simulink model "IPMSMVelocityControl"  (R2024a)
settings: Solver=FixedStepDiscrete  StartTime=0.0  StopTime=1  FixedStep=Ts  RelTol=1e-3  EnableMultiTasking=on
PreLoadFcn:
  | IPMSMVelocityControlData;
undefined symbols (not defined in the file): Ld, Lq, p, psim, Ts, VDC_VECT
libraries: nesl_utility x13, fl_lib x10, ee_lib x4, eeTransforms x2, batteryecm_lib x1, eePmsmCurrentController x1, simulink x1, eePmsmCurrentReferenceGen x1, eeVelocityController x1, eePwmGeneratorTwoLevel x1, SignalEditorBlockLib x1
CloseFcn:
  | try,close(h1_IPMSMVelocityControl),end
  | clear h1_IPMSMVelocityControl
  | 
  | clear simlog_IPMSMVelocityControl
  | clear logsout_IPMSMVelocityControl
  | 
  | clear Pmax Tmax p psim Ld Lq L0 Rs Jm
  | clear Cdc Vnom V1 AH0
  | clear Ts fsw Tsi Tso Kp_id Ki_id Kp_iq Ki_iq
  | clear numd_id dend_id numd_iq dend_iq
  | clear Kp_omega Ki_omega numd_omega dend_omega
  | clear ID_MAP IQ_MAP RPM_VECT TQ_VECT VDC_VECT
Description:
  | IPMSM Velocity Control
settings Model: Creator=The MathWorks, Inc.  LastModifiedBy=hirah
settings SolverCC: AlgebraicLoopSolver=TrustRegion  MaxZcPerStep=1
settings DataIOCC: MaxDataPoints=210000  ReturnWorkspaceOutputs=off  SignalLoggingName=logsout_IPMSMVelocityControl
settings OptimizationCC: ReuseModelBlockBuffer=off  LifeSpan=inf
settings DebuggingCC: UnderspecifiedInitializationDetection=Classic  MergeDetectMultiDrivingBlocksExec=none  UnconnectedInputMsg=warning  UnconnectedOutputMsg=warning  UnconnectedLineMsg=warning  SFUnexpectedBacktrackingDiag=warning  SFNoUnconditionalDefaultTransitionDiag=warning  SFExecutionAtInitializationDiag=none  ArithmeticOperatorsInVariantConditions=warning
settings ModelReferenceCC: EnableRefExpFcnMdlSchedulingChecks=on
settings SFSimCC: SimUseLocalCustomCode=off  CustomCodeUndefinedFunction=UseInterfaceOnly
settings RTWCC: RTWUseLocalCustomCode=off  GPUComputeCapability=3.5  DLArmComputeVersion=19.05
settings CodeAppCC: StateflowObjectComments=on
settings GRTTargetCC: TargetLangStandard=C89/C90 (ANSI)
settings ConfigComp: CovMetricSettings=dw  CovSaveCumulativeToWorkspaceVar=on  CovSaveSingleToWorkspaceVar=on  CovExternalEMLEnable=off
settings SimscapeCC: SimscapeNormalizeSystem=off  SimscapeLogType=all  SimscapeLogSimulationStatistics=on  SimscapeLogName=simlog_IPMSMVelocityControl  SimscapeLogDataHistory=210000

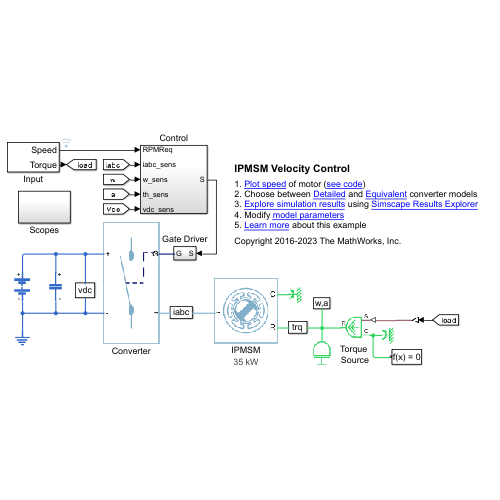
[thumbnail: Simulink's stored preview of the top-level diagram]
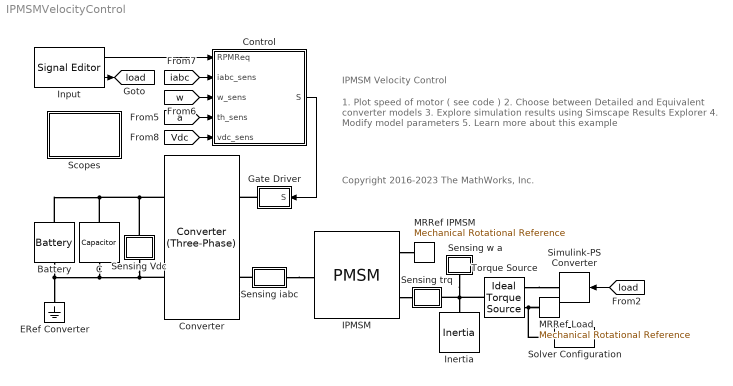
== system IPMSMVelocityControl ==
  note: IPMSM Velocity Control
  note: 1. Plot speed of motor ( see code )
      | 2. Choose between Detailed and Equivalent converter models
      | 3. Explore simulation results using Simscape Results Explorer
      | 4. Modify model parameters
      | 5. Learn more about this example
  note: Copyright 2016-2023 The MathWorks, Inc.
  Battery : batteryecm_lib/Battery  Vnom=Vnom V  prm_dir=1  R1_dis=2 Ohm  R1_ch=2 Ohm  R1=0.001 Ohm  prm_AH=1  AH=300 hr*A  V1=V1 V  AH1=100 hr*A  prm_R2=1  R2=2000 Ohm  Tmeas=298.15 K  charge_measurement_port=simscape.enum.battery.enable.no  prm_dyn=1  Rp1=0.005 Ohm  tau1=30 s  Rp2=0.005 Ohm  tau2=30 s  Rp3=0.005 Ohm  tau3=30 s  Rp4=0.005 Ohm  tau4=30 s  Rp5=0.005 Ohm  tau5=30 s  prm_fade=1  N_fade=100  AH_fade=45 hr*A  R1_fade=2.02 Ohm  R1_ch_fade=2.02 Ohm  V1_fade=10.35 V  prm_age=1  prm_age_OCV=1  OCV_age=0.9  SOC_age=60  Tmeas_age=298.15 K  delta_time_age_vec=[0] d  temperature_age_vec=[273] K  OCV_scaling_age=2.2134e6  OCV_offset_age=1.632e6  temp_exp_age=0.515833569 V  t_exp_age=0.75  Vnom_T2=12 V  R1_T2=2.2 Ohm  R1_T2_dis=2.2 Ohm  R1_T2_ch=2.2 Ohm  V1_T2=11.4 V  R2_T2=2200 Ohm  Rp1_T2=0.005 Ohm  tau1_T2=30 s  Rp2_T2=0.005 Ohm  tau2_T2=30 s  Rp3_T2=0.005 Ohm  tau3_T2=30 s  Rp4_T2=0.005 Ohm  tau4_T2=30 s  Rp5_T2=0.005 Ohm  tau5_T2=30 s  Tmeas2=273.15 K  thermal_port=simscape.enum.thermaleffects.omit  thermal_mass=30000 J/K  i_specify=off  i_priority=None  i=0 A  i_nominal_specify=off  i_nominal_value=1  i_nominal_unit=A  v_specify=off  v_priority=None  v=0 V  v_nominal_specify=off  v_nominal_value=1  v_nominal_unit=V  charge_specify=on  charge_priority=High  charge=AH0 hr*A  charge_nominal_specify=off  charge_nominal_value=1  charge_nominal_unit=A*hr  num_cycles_specify=off  num_cycles_priority=High  num_cycles=0  num_cycles_nominal_specify=off  num_cycles_nominal_value=1  num_cycles_nominal_unit=1  temperature_specify=off  temperature_priority=High  temperature=298.15 K  temperature_nominal_specify=off  temperature_nominal_value=1  temperature_nominal_unit=K
  C : fl_lib/Electrical/Electrical Elements/Capacitor  c=Cdc F  r=1e-6 Ohm  g=0 1/Ohm  i_specify=off  i_priority=None  i=0 A  i_nominal_specify=off  i_nominal_value=1  i_nominal_unit=A  v_specify=off  v_priority=None  v=0 V  v_nominal_specify=off  v_nominal_value=1  v_nominal_unit=V  vc_specify=on  vc_priority=None  vc=Vnom V  vc_nominal_specify=off  vc_nominal_value=1  vc_nominal_unit=V
  Control : Subsystem
  Converter : ee_lib/Semiconductors & Converters/Converters/Converter (Three-Phase)  port_option=ee.enum.threePhasePort.composite  fidelity_option=ee.enum.converters.fidelity.detailed  device_type=3  K=0  Vf=0.8 V  Ron=0.001 Ohm  Rds=0.001 Ohm  Goff=1e-5 1/Ohm  Vgt=1 V  Vgt_off=-1 V  Ih=1 A  Vth=0.5 V  diode_param=2  diode_Vf=0.8 V  diode_Ron=0.001 Ohm  diode_Goff=1e-5 1/Ohm  diode_C=50 nF  diode_iRM=-235 A  diode_iF=300 A  diode_idot=-50 A/us  diode_trr_param=1  diode_trr_factor=3  diode_trr=15 us  diode_Qrr=1.5e+3 s*uA  snubber_type=0  Cs=1e-7 F  Rs=0.1 Ohm
  ERef Converter : fl_lib/Electrical/Electrical Elements/Electrical Reference
  Gate Driver : Subsystem
  IPMSM : ee_lib/Electromechanical/Permanent Magnet/PMSM  port_option=ee.enum.threePhasePort.composite  winding_type=ee.enum.statorconnection.wye  machine_param=ee.enum.pmsm.parameterization.constant  nPolePairs=p  pmflux_param=1  pm_flux_linkage=psim Wb  torque_constant=0.18 N*m/A  back_emf_constant=0.18 V/(rad/s)  stator_param=1  Ld=Ld H  Lq=Lq H  idVec=[-200, 0, 200] A  iqVec=[-200, 0, 200] A  LdMatrix=0.0002 * ones(3, 3) H  LqMatrix=0.0002 * ones(3, 3) H  PmMatrix=0.1 * ones(3, 3) Wb  ktMatrix=0.18 * ones(3, 3) N*m/A  keMatrix=0.18 * ones(3, 3) V/(rad/s)  L0=L0 H  Ls=0.0002 H  Lm=0.00002 H  Ms=0.00002 H  Rs=Rs Ohm  zero_sequence=ee.enum.park.zerosequence.exclude  axes_param=1  loss_param=ee.enum.ironloss.none  losses_oc=[0, 0, 0] W  losses_sc=[0, 0, 0] W  f_losses=60 Hz  Isc_losses=95 A  J=0 kg*m^2  lam=0 N*m/(rad/s)  i_d_specify=off  i_d_priority=None  i_d=0 A  i_d_nominal_specify=off  i_d_nominal_value=1  i_d_nominal_unit=A  i_q_specify=off  i_q_priority=None  i_q=0 A  i_q_nominal_specify=off  i_q_nominal_value=1  i_q_nominal_unit=A  torque_specify=off  torque_priority=None  torque=0 N*m  torque_nominal_specify=off  torque_nominal_value=1  torque_nominal_unit=N*m  angular_velocity_specify=on  angular_velocity_priority=None  angular_velocity=0 rpm  angular_velocity_nominal_specify=off  angular_velocity_nominal_value=1  angular_velocity_nominal_unit=rpm  angular_position_specify=on  angular_position_priority=High  angular_position=0 rad  angular_position_nominal_specify=off  angular_position_nominal_value=1  angular_position_nominal_unit=deg  alpha=3.93e-3 1/K  alpha_flux=-0.001 1/K  Tmeas=298.15 K  stator_thermal_mass=100 J/K  rotor_thermal_mass=200 J/K  Rm_percent_rotor=90  Rd_percent_rotor=30  temperatureA_specify=off  temperatureA_priority=High  temperatureA=25 degC  temperatureA_nominal_specify=off  temperatureA_nominal_value=1  temperatureA_nominal_unit=degC  temperatureB_specify=off  temperatureB_priority=High  temperatureB=25 degC  temperatureB_nominal_specify=off  temperatureB_nominal_value=1  temperatureB_nominal_unit=degC  temperatureC_specify=off  temperatureC_priority=High  temperatureC=25 degC  temperatureC_nominal_specify=off  temperatureC_nominal_value=1  temperatureC_nominal_unit=degC  temperatureR_specify=off  temperatureR_priority=High  temperatureR=25 degC  temperatureR_nominal_specify=off  temperatureR_nominal_value=1  temperatureR_nominal_unit=degC
      settings: AttributesFormatString=35 kW  InternalSimscapePortConfiguration="{\"Bottom\":[],\"Left\":[{\"id\":\"N\",\"label\":\"~\",\"type\":\"foundation.electrical.three_phase\"}],\"Right\":[{\"id\":\"R\",\"label\":\"R\",\"type\":\"foundation.mechanical.rotational.rotational\"},{\"id\":\"C\",\"label\":\"C\",\"type\":\"foundation.mechanical.rotational.rotational\"}],\"Top\":[]}"
  Inertia : fl_lib/Mechanical/Rotational Elements/Inertia  inertia=Jm kg*m^2  num_ports=foundation.enum.numPorts2.one  w_specify=on  w_priority=High  w=0 rpm  w_nominal_specify=off  w_nominal_value=1  w_nominal_unit=rad/s  t_specify=off  t_priority=High  t=0 N*m  t_nominal_specify=off  t_nominal_value=1  t_nominal_unit=N*m
  Input : SignalEditorBlockLib/Signal Editor  FileName=IPMSMVelocityControlInput.mat  ActiveScenario=Test_1  ActiveSignal=Torque  IsBus=off  OutputBusObjectStr=Bus: BusObject  SampleTime=0  OutputAfterFinalValue=Extrapolation  Unit=inherit  PreserveSignalName=on  ApplySigPropsToAllScenarios=on  ApplySigPropsToAllSignals=off
  MRRef IPMSM : fl_lib/Mechanical/Rotational Elements/Mechanical Rotational Reference
  MRRef Load : fl_lib/Mechanical/Rotational Elements/Mechanical Rotational Reference
  Scopes : Subsystem
  Sensing Vdc : Subsystem
      mask Display: disp('vdc')
  Sensing trq : Subsystem
      mask Display: disp('trq')
  Sensing w a : Subsystem
      mask Display: disp('w,a')
  Sensing iabc : Subsystem
      mask Display: disp('iabc')
  Simulink-PS Converter : nesl_utility/Simulink-PS Converter  PhysicalDomain=network_engine_domain  SubClassName=ps_input  LeftPortType=input  RightPortType=output  PseudoPeriodic=off  Frequencies=[]  NoiseDistribution=none  NoiseParameters=[]  Unit=N*m  AffineConversion=off  FilteringAndDerivatives=zero  SimscapeFilterOrder=1  InputFilterTimeConstant=0.001  UdotUserProvided=1
  Solver Configuration : nesl_utility/Solver Configuration  PhysicalDomain=network_engine_domain  SubClassName=solver  LeftPortType=input  RightPortType=generic  Tones=[]  Harmonics=[]  SimulateNoise=off  Profile=off  UseLocalSampling=off  EnableSwitchedLinearOptims=on  FrequencyDomain=off  UseCCode=off  RelTol=0.001  AbsTol=1e-06  MinStep=1e-09  ToWorkspace=off  RevertToSquareIcSolve=off  NumHomotopyIterations=100  PhasorMode=off  PhasorModeNumHarmonics=1  ConsistencySolver=NEWTON_FTOL  IndexReductionMethod=DerivativeReplacement  DoDC=off  ResidualTolerance=1e-9  ConsistencyTolSource=GLOBAL  ConsistencyAbsTol=0.001  ConsistencyRelTol=0.001  ConsistencyTolFactor=0.001  UseLocalSolver=on  LocalSolverChoice=NE_BACKWARD_EULER_ADVANCER  ResolveIndetEquations=on  FunctionEvalNumThread=1  LocalSolverSampleTime=Ts  DoFixedCost=on  MaxNonlinIter=5  MaxModeIter=2  ComputeImpulses=off  ImpulseIterations=2  LinearAlgebra=auto  LinearAlgebraNumThread=0  EquationFormulation=NE_TIME_EF  DelaysMemoryBudget=1024  AutomaticFiltering=on  FilteringTimeConstant=0.001  PartitionStorageMethod=AS_NEEDED  PartitionMemoryBudget=1024  PartitionMethod=FAST  MultibodyUseLocalSolver=off  MultibodyLocalSolverChoice=ODE1  MultibodyLocalSolverSampleTime=0.001
  Torque Source : fl_lib/Mechanical/Mechanical Sources/Ideal Torque Source
  tag scope: load=global
  wires:
  Control/1(S) -> Gate Driver/1(S)
  [load] -> Simulink-PS Converter/1
  Input/1 -> Control/1(RPMReq)
  [Vdc] -> Control/5(vdc_sens)
  [iabc] -> Control/2(iabc_sens)
  [w] -> Control/3(w_sens)
  [a] -> Control/4(th_sens)
  Input/2 -> [load]
  connections:
  Converter/RConn1 -- Sensing Vdc/LConn1 -- Battery/LConn1 -- C/LConn1
  Torque Source/LConn1 -- Sensing trq/RConn1 -- Inertia/LConn1 -- Sensing w a/LConn1
  Gate Driver/RConn1 -- Converter/LConn1
  Torque Source/RConn1 -- Simulink-PS Converter/RConn1
  Torque Source/RConn2 -- Solver Configuration/RConn1 -- MRRef Load/LConn1
  Sensing iabc/LConn1 -- Converter/LConn2
  Sensing iabc/RConn1 -- IPMSM/LConn1
  IPMSM/RConn2 -- MRRef IPMSM/LConn1
  IPMSM/RConn1 -- Sensing trq/LConn1
  Battery/RConn1 -- Converter/RConn2 -- Sensing Vdc/RConn1 -- C/RConn1 -- ERef Converter/LConn1

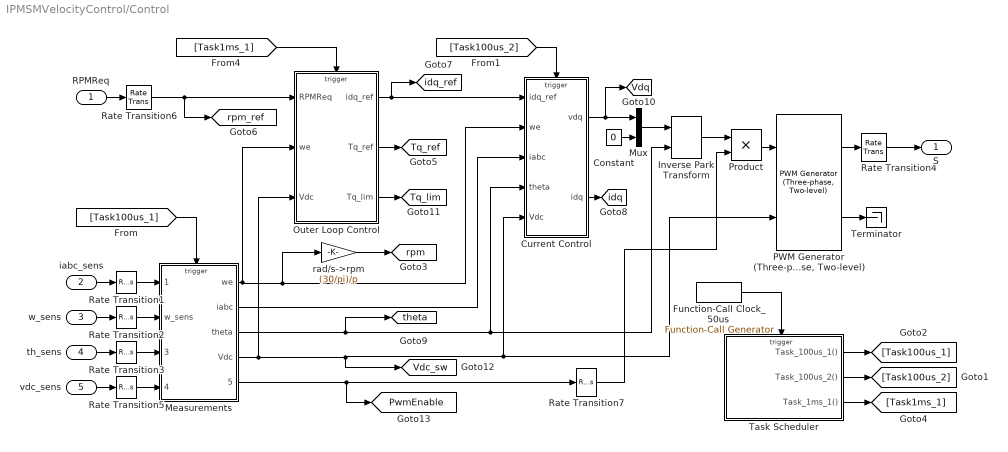
== system IPMSMVelocityControl/Control ==
  RPMReq : Inport
  iabc_sens : Inport  Port=2
  w_sens : Inport  Port=3
  th_sens : Inport  Port=4
  vdc_sens : Inport  Port=5
  Constant : Constant  Value=0  SampleTime=-1
  Current Control : Subsystem
  Function-Call Clock_50us : simulink/Ports & Subsystems/Function-Call Generator  sample_time=5e-5  numberOfIterations=1  DisallowWideOutput=off
  Inverse Park Transform : eeTransforms/Inverse Park Transform  AxisAlignment=Q-axis  PowerInvariant=off
  Measurements : Subsystem
  Mux : Mux  Inputs=2
  Outer Loop Control : Subsystem
  "PWM Generator (Three-phase, Two-level)" : eePwmGeneratorTwoLevel/PWM Generator (Three-phase, Two-level)  PWMMode=Continuous PWM (CPWM)  CPWMMode=SVM: space vector modulation  DPWMMode=60 DPWM: 60 degree discontinuous PWM  fsw=fsw  Ts=Ts
  Product : Product
  Rate Transition{1..7} (7 alike) : RateTransition
  Task Scheduler : Stateflow chart  TreatAsAtomicUnit=on
  Terminator : Terminator
  rad/s->rpm : Gain  Gain=(30/pi)/p
  S : Outport  VectorParamsAs1DForOutWhenUnconnected=off
  tag scope: PwmEnable=global, Tq_lim=global, Tq_ref=global, Vdc_sw=global, Vdq=global, idq=global, idq_ref=global, rpm=global, rpm_ref=global, theta=global
  wires:
  [Task100us_1] -> Measurements/Trigger
  [Task100us_2] -> Current Control/Trigger
  Current Control/1(vdq) -> Mux/1, [Vdq]
  Measurements/2(iabc) -> Current Control/3(iabc)
  Measurements/3(theta) -> [theta], Current Control/4(theta), Inverse Park Transform/2
  "PWM Generator (Three-phase, Two-level)"/1 -> Rate Transition4/1
  iabc_sens/1 -> Rate Transition1/1
  w_sens/1 -> Rate Transition2/1
  th_sens/1 -> Rate Transition3/1
  vdc_sens/1 -> Rate Transition5/1
  Outer Loop Control/1(idq_ref) -> [idq_ref], Current Control/1(idq_ref)
  RPMReq/1 -> Rate Transition6/1
  "PWM Generator (Three-phase, Two-level)"/2 -> Terminator/1
  Rate Transition1/1 -> Measurements/1(iabc_sens)
  Rate Transition2/1 -> Measurements/2(w_sens)
  Rate Transition3/1 -> Measurements/3(th_sens)
  Rate Transition5/1 -> Measurements/4(Vdc_sens)
  Rate Transition6/1 -> [rpm_ref], Outer Loop Control/1(RPMReq)
  Measurements/4(Vdc) -> [Vdc_sw], Current Control/5(Vdc), "PWM Generator (Three-phase, Two-level)"/2, Outer Loop Control/3(Vdc)
  Function-Call Clock_50us/1 -> Task Scheduler/Trigger
  Task Scheduler/3(Task_1ms_1()) -> [Task1ms_1]
  Task Scheduler/2(Task_100us_2()) -> [Task100us_2]
  Task Scheduler/1(Task_100us_1()) -> [Task100us_1]
  Outer Loop Control/2(Tq_ref) -> [Tq_ref]
  Measurements/1(we) -> Current Control/2(we), rad/s->rpm/1, Outer Loop Control/2(we)
  rad/s->rpm/1 -> [rpm]
  Current Control/2(idq) -> [idq]
  Outer Loop Control/3(Tq_lim) -> [Tq_lim]
  Measurements/5(PwmEnable) -> [PwmEnable], Rate Transition7/1
  [Task1ms_1] -> Outer Loop Control/Trigger
  Mux/1 -> Inverse Park Transform/1
  Constant/1 -> Mux/2
  Rate Transition4/1 -> S/1
  Product/1 -> "PWM Generator (Three-phase, Two-level)"/1
  Inverse Park Transform/1 -> Product/1
  Rate Transition7/1 -> Product/2

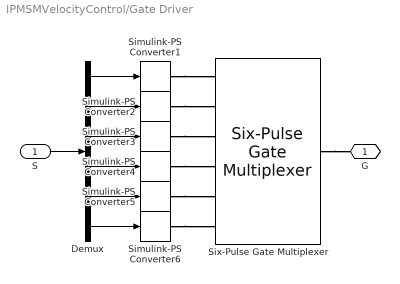
== system IPMSMVelocityControl/Gate Driver ==
  S : Inport
  Demux : Demux  Outputs=6
  Simulink-PS Converter{1..6} (6 alike) : nesl_utility/Simulink-PS Converter  PhysicalDomain=network_engine_domain  SubClassName=ps_input  LeftPortType=input  RightPortType=output  PseudoPeriodic=off  Frequencies=[]  NoiseDistribution=none  NoiseParameters=[]  Unit=1  AffineConversion=off  FilteringAndDerivatives=zero  SimscapeFilterOrder=1  InputFilterTimeConstant=0.001  UdotUserProvided=1
  Six-Pulse Gate Multiplexer : ee_lib/Semiconductors & Converters/Converters/Six-Pulse Gate Multiplexer  port_option=ee.enum.controlport.ps
  G : PMIOPort  Side=Right
  wires:
  Demux/1 -> Simulink-PS Converter1/1
  S/1 -> Demux/1
  Demux/4 -> Simulink-PS Converter4/1
  Demux/2 -> Simulink-PS Converter2/1
  Demux/3 -> Simulink-PS Converter3/1
  Demux/5 -> Simulink-PS Converter5/1
  Demux/6 -> Simulink-PS Converter6/1
  connections:
  Six-Pulse Gate Multiplexer/RConn1 -- G/RConn1
  Simulink-PS Converter1/RConn1 -- Six-Pulse Gate Multiplexer/LConn1
  Simulink-PS Converter3/RConn1 -- Six-Pulse Gate Multiplexer/LConn3
  Simulink-PS Converter5/RConn1 -- Six-Pulse Gate Multiplexer/LConn5
  Simulink-PS Converter6/RConn1 -- Six-Pulse Gate Multiplexer/LConn6
  Simulink-PS Converter4/RConn1 -- Six-Pulse Gate Multiplexer/LConn4
  Simulink-PS Converter2/RConn1 -- Six-Pulse Gate Multiplexer/LConn2

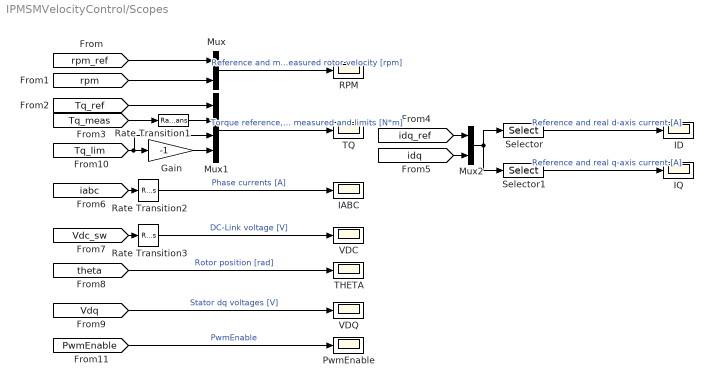
== system IPMSMVelocityControl/Scopes ==
  Gain : Gain  Gain=-1
  IABC : Scope
  ID : Scope
  IQ : Scope
  Mux : Mux  Inputs=2
  Mux1 : Mux
  Mux2 : Mux  Inputs=2
  PwmEnable : Scope
  RPM : Scope
  Rate Transition1 : RateTransition
  Rate Transition2 : RateTransition  OutPortSampleTime=1e-4
  Rate Transition3 : RateTransition  OutPortSampleTime=1e-4
  Selector : Selector  InputPortWidth=4  IndexOptions=Index vector (dialog)  Indices=[1 3]  OutputSizes=1
  Selector1 : Selector  InputPortWidth=4  IndexOptions=Index vector (dialog)  Indices=[2 4]  OutputSizes=1
  THETA : Scope
  TQ : Scope
  VDC : Scope
  VDQ : Scope
  wires:
  [rpm] -> Mux/2
  Selector1/1 -> IQ/1  "Reference and real q-axis current [A]"
  Mux2/1 -> Selector1/1, Selector/1
  Gain/1 -> Mux1/4
  Rate Transition3/1 -> VDC/1  "DC-Link voltage [V]"
  [Vdc_sw] -> Rate Transition3/1
  [idq_ref] -> Mux2/1
  [PwmEnable] -> PwmEnable/1  "PwmEnable"
  [Tq_ref] -> Mux1/1
  Rate Transition2/1 -> IABC/1  "Phase currents [A]"
  [idq] -> Mux2/2
  [rpm_ref] -> Mux/1
  [iabc] -> Rate Transition2/1
  [Tq_meas] -> Rate Transition1/1
  [Vdq] -> VDQ/1  "Stator dq voltages [V]"
  Selector/1 -> ID/1  "Reference and real d-axis current [A]"
  [Tq_lim] -> Mux1/3, Gain/1
  Mux1/1 -> TQ/1  "Torque reference, measured and limits [N*m]"
  [theta] -> THETA/1  "Rotor position [rad]"
  Rate Transition1/1 -> Mux1/2
  Mux/1 -> RPM/1  "Reference and measured rotor velocity [rpm]"

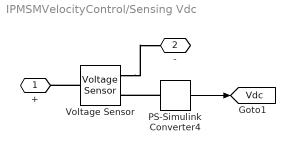
== system IPMSMVelocityControl/Sensing Vdc ==
  PS-Simulink Converter4 : nesl_utility/PS-Simulink Converter  PhysicalDomain=network_engine_domain  SubClassName=ps_output  LeftPortType=input  RightPortType=output  PseudoPeriodic=off  Frequencies=[]  VectorFormat=1-D array  Unit=V  AffineConversion=off
  Voltage Sensor : fl_lib/Electrical/Electrical Sensors/Voltage Sensor
  + : PMIOPort  Side=Left
  - : PMIOPort  Port=2  Side=Right
  tag scope: Vdc=global
  wires:
  PS-Simulink Converter4/1 -> [Vdc]
  connections:
  Voltage Sensor/LConn1 -- +/RConn1
  Voltage Sensor/RConn2 -- -/RConn1
  PS-Simulink Converter4/LConn1 -- Voltage Sensor/RConn1

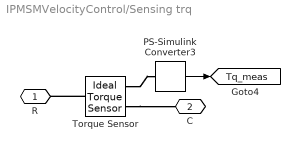
== system IPMSMVelocityControl/Sensing trq ==
  PS-Simulink Converter3 : nesl_utility/PS-Simulink Converter  PhysicalDomain=network_engine_domain  SubClassName=ps_output  LeftPortType=input  RightPortType=output  PseudoPeriodic=off  Frequencies=[]  VectorFormat=1-D array  Unit=N*m  AffineConversion=off
  Torque Sensor : fl_lib/Mechanical/Mechanical Sensors/Ideal Torque Sensor
  R : PMIOPort  Side=Left
  C : PMIOPort  Port=2  Side=Right
  tag scope: Tq_meas=global
  wires:
  PS-Simulink Converter3/1 -> [Tq_meas]
  connections:
  Torque Sensor/RConn1 -- C/RConn1
  Torque Sensor/RConn2 -- PS-Simulink Converter3/LConn1
  Torque Sensor/LConn1 -- R/RConn1

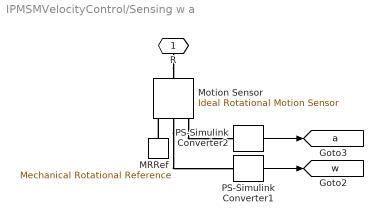
== system IPMSMVelocityControl/Sensing w a ==
  MRRef : fl_lib/Mechanical/Rotational Elements/Mechanical Rotational Reference
  Motion Sensor : fl_lib/Mechanical/Mechanical Sensors/Ideal Rotational Motion Sensor  reference=foundation.enum.MeasurementReference.difference  acceleration_port=false  velocity_port=true  position_port=true  wrap_angle=simscape.enum.onoff.off  offset=0 deg
  PS-Simulink Converter1 : nesl_utility/PS-Simulink Converter  PhysicalDomain=network_engine_domain  SubClassName=ps_output  LeftPortType=input  RightPortType=output  PseudoPeriodic=off  Frequencies=[]  VectorFormat=1-D array  Unit=rad/s  AffineConversion=off
  PS-Simulink Converter2 : nesl_utility/PS-Simulink Converter  PhysicalDomain=network_engine_domain  SubClassName=ps_output  LeftPortType=input  RightPortType=output  PseudoPeriodic=off  Frequencies=[]  VectorFormat=1-D array  Unit=rad  AffineConversion=off
  R : PMIOPort  Side=Left
  tag scope: a=global, w=global
  wires:
  PS-Simulink Converter1/1 -> [w]
  PS-Simulink Converter2/1 -> [a]
  connections:
  R/RConn1 -- Motion Sensor/LConn1
  Motion Sensor/RConn2 -- PS-Simulink Converter1/LConn1
  MRRef/LConn1 -- Motion Sensor/RConn1
  Motion Sensor/RConn3 -- PS-Simulink Converter2/LConn1

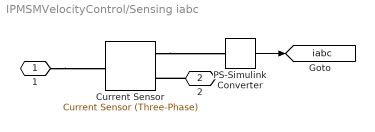
== system IPMSMVelocityControl/Sensing iabc ==
  Current Sensor : ee_lib/Sensors & Transducers/Current Sensor (Three-Phase)
  PS-Simulink Converter : nesl_utility/PS-Simulink Converter  PhysicalDomain=network_engine_domain  SubClassName=ps_output  LeftPortType=input  RightPortType=output  PseudoPeriodic=off  Frequencies=[]  VectorFormat=1-D array  Unit=A  AffineConversion=off
  1 : PMIOPort  Side=Left
  2 : PMIOPort  Port=2  Side=Right
  tag scope: iabc=global
  wires:
  PS-Simulink Converter/1 -> [iabc]
  connections:
  1/RConn1 -- Current Sensor/LConn1
  2/RConn1 -- Current Sensor/RConn2
  Current Sensor/RConn1 -- PS-Simulink Converter/LConn1

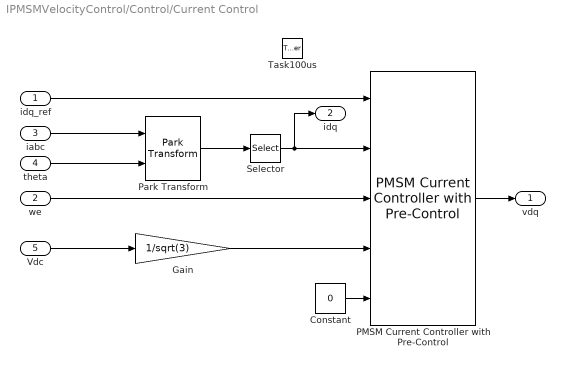
== system IPMSMVelocityControl/Control/Current Control ==
  idq_ref : Inport
  we : Inport  Port=2
  iabc : Inport  Port=3
  theta : Inport  Port=4
  Vdc : Inport  Port=5
  Task100us : TriggerPort  TriggerType=function-call  VariantControl=Variant  PortDimensions=1
  Constant : Constant  Value=0  SampleTime=-1
  Gain : Gain  Gain=1/sqrt(3)
  PMSM Current Controller with Pre-Control : eePmsmCurrentController/PMSM Current Controller with Pre-Control  Kp_id=Kp_id  Ki_id=Ki_id  Kaw_id=1  Kp_iq=Kp_iq  Ki_iq=Ki_iq  Kaw_iq=1  Ts=-1  Tsd=Tsi  AxisPrio=Q-axis  ActZC=on  ActFF=on  idVect=[-200, 0, 200]  iqVect=[-200, 0, 200]  LdMatrix=Ld * ones(3, 3)  LqMatrix=Lq * ones(3, 3)  psimMatrix=psim * ones(3, 3)
  Park Transform : eeTransforms/Park Transform  AxisAlignment=Q-axis  PowerInvariant=off
  Selector : Selector  InputPortWidth=3  IndexOptions=Index vector (dialog)  Indices=[1 2]  OutputSizes=1
  vdq : Outport  VectorParamsAs1DForOutWhenUnconnected=off
  idq : Outport  Port=2  VectorParamsAs1DForOutWhenUnconnected=off
  wires:
  Vdc/1 -> Gain/1
  iabc/1 -> Park Transform/1
  we/1 -> PMSM Current Controller with Pre-Control/3
  theta/1 -> Park Transform/2
  PMSM Current Controller with Pre-Control/1 -> vdq/1
  idq_ref/1 -> PMSM Current Controller with Pre-Control/1
  Constant/1 -> PMSM Current Controller with Pre-Control/5
  Selector/1 -> idq/1, PMSM Current Controller with Pre-Control/2
  Gain/1 -> PMSM Current Controller with Pre-Control/4
  Park Transform/1 -> Selector/1

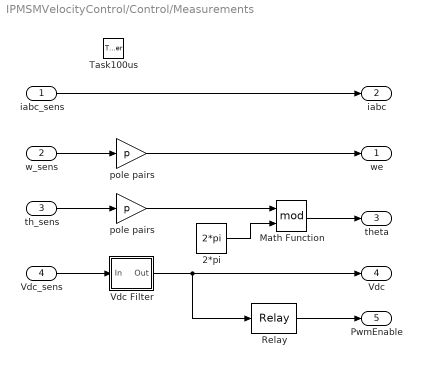
== system IPMSMVelocityControl/Control/Measurements ==
  iabc_sens : Inport
  w_sens : Inport  Port=2
  th_sens : Inport  Port=3
  Vdc_sens : Inport  Port=4
  Task100us : TriggerPort  TriggerType=function-call  VariantControl=Variant  PortDimensions=1
  2*pi : Constant  Value=2*pi  SampleTime=-1
  Math Function : Math  Operator=mod  SignedPower=on
  Relay : Relay  OnSwitchValue=VDC_VECT(1)  OffSwitchValue=0.5*VDC_VECT(1)
  Vdc Filter : Subsystem  mask(Discrete first-order filter (Low-pass)){T=0.005, Ts=1e-4}
      mask prompts: T "Time constant (s):"; Ts "Sample time (s):"
      mask help: This block implements a discrete low-pass filter. To calculate the coefficients, the block discretises a continuous low-pass filter using the Tustin method.
      mask init:
      | num = [ Ts/(2*T + Ts), Ts/(2*T + Ts)];
      | den = [ 1, -(2*T - Ts)/(2*T + Ts)];
  pole pairs : Gain  Gain=p
  "pole pairs " : Gain  Gain=p
  we : Outport  VectorParamsAs1DForOutWhenUnconnected=off
  iabc : Outport  Port=2  VectorParamsAs1DForOutWhenUnconnected=off
  theta : Outport  Port=3  VectorParamsAs1DForOutWhenUnconnected=off
  Vdc : Outport  Port=4  VectorParamsAs1DForOutWhenUnconnected=off
  PwmEnable : Outport  Port=5  VectorParamsAs1DForOutWhenUnconnected=off
  wires:
  pole pairs/1 -> we/1
  Vdc_sens/1 -> Vdc Filter/1(In)
  th_sens/1 -> "pole pairs "/1
  w_sens/1 -> pole pairs/1
  iabc_sens/1 -> iabc/1
  "pole pairs "/1 -> Math Function/1
  2*pi/1 -> Math Function/2
  Math Function/1 -> theta/1
  Relay/1 -> PwmEnable/1
  Vdc Filter/1(Out) -> Relay/1, Vdc/1

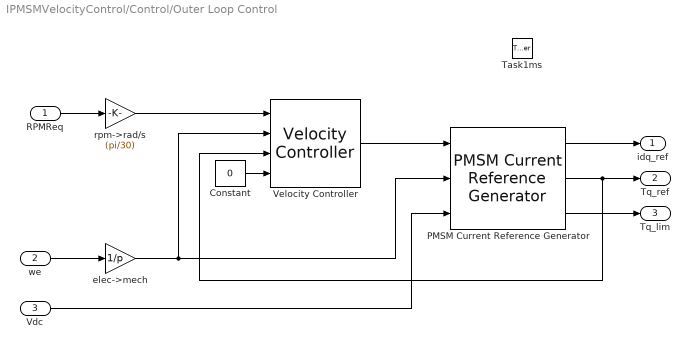
== system IPMSMVelocityControl/Control/Outer Loop Control ==
  RPMReq : Inport
  we : Inport  Port=2
  Vdc : Inport  Port=3
  Task1ms : TriggerPort  TriggerType=function-call  VariantControl=Variant  PortDimensions=1
  Constant : Constant  Value=0  SampleTime=-1
  PMSM Current Reference Generator : eePmsmCurrentReferenceGen/PMSM Current Reference Generator  Vnom=Vnom  Pmax=Pmax  Tmax=Tmax  Ts=-1  RefType=Lookup-table based  rpmVec=RPM_VECT  TqVec=TQ_VECT  VdcVec=VDC_VECT  PWMMode=SVM: space vector modulation  ModFactor=1  idMatrix=ID_MAP  iqMatrix=IQ_MAP  p=8  psim=0.04  Ld=0.00024  Lq=0.00029  Rs=0.01  RefExpEnable=0
  Velocity Controller : eeVelocityController/Velocity Controller  CtrlType=P-PI control  Kp_w=Kp_omega  Ki_w=Ki_omega  Kv_w=Kp_omega  Kaw_w=100  Ts=-1  Tsd=Tso  ActZC=on
  elec->mech : Gain  Gain=1/p
  rpm->rad/s : Gain  Gain=(pi/30)
  idq_ref : Outport  VectorParamsAs1DForOutWhenUnconnected=off
  Tq_ref : Outport  Port=2  VectorParamsAs1DForOutWhenUnconnected=off
  Tq_lim : Outport  Port=3  VectorParamsAs1DForOutWhenUnconnected=off
  wires:
  rpm->rad/s/1 -> Velocity Controller/1
  Velocity Controller/1 -> PMSM Current Reference Generator/1
  RPMReq/1 -> rpm->rad/s/1
  we/1 -> elec->mech/1
  Vdc/1 -> PMSM Current Reference Generator/3
  PMSM Current Reference Generator/1 -> idq_ref/1
  PMSM Current Reference Generator/2 -> Tq_ref/1, Velocity Controller/3
  PMSM Current Reference Generator/3 -> Tq_lim/1
  elec->mech/1 -> PMSM Current Reference Generator/2, Velocity Controller/2
  Constant/1 -> Velocity Controller/4

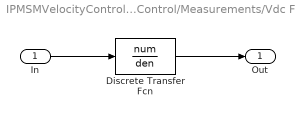
== system IPMSMVelocityControl/Control/Measurements/Vdc Filter ==
  In : Inport
  Discrete Transfer Fcn : DiscreteTransferFcn  Numerator=num  Denominator=den
  Out : Outport  VectorParamsAs1DForOutWhenUnconnected=off
  wires:
  Discrete Transfer Fcn/1 -> Out/1
  In/1 -> Discrete Transfer Fcn/1

== stateflow chart IPMSMVelocityControl/Control/Task Scheduler ==
  (default) -> (junction 23) : CLK_50us
  (junction 23) -> (junction 17)
  (junction 17) -> (junction 22) [order 2]
  (junction 17) -> (junction 22) [order 1] : [cnt%%2==0]{Task_100us_1;}
  (junction 22) -> (junction 18) [order 2]
  (junction 22) -> (junction 18) [order 1] : [cnt%%2==0]{Task_100us_2;}
  (junction 18) -> (junction 21) [order 1] : [cnt%%20==0]{Task_1ms_1;}
  (junction 18) -> (junction 21) [order 2]
  (junction 21) -> (junction 34) [order 2]
  (junction 21) -> (junction 16) [order 1] : [1]{cnt++;}
  data: cnt local int32
  events: Task_100us_1 output FUNCTION_CALL_EVENT; Task_100us_2 output FUNCTION_CALL_EVENT; Task_1ms_1 output FUNCTION_CALL_EVENT; CLK_50us input FUNCTION_CALL_EVENT
